simulink model "sm_pump_triplex"  (R2025a)
settings: Solver=VariableStepAuto  StartTime=0.0  StopTime=1.5  RelTol=1e-3  EnableMultiTasking=on
undefined symbols (not defined in the file): pOut_Init_WKSP, smiData, TRP_Par, X, Y, Z
libraries: sm_lib x43, fl_lib x30, nesl_utility x11, simulink x10, SimscapeFluids_lib x3, sm_pump_triplex_lib x3, ee_lib x2, Multibody_Multiphysics_Lib x1
(part 1 of 3)
CloseFcn:
  | try,close(h1_sm_pump_triplex),end
  | clear h1_sm_pump_triplex
  | try,close(h2_sm_pump_triplex),end
  | clear h2_sm_pump_triplex
  | try,close(h3_sm_pump_triplex),end
  | clear h3_sm_pump_triplex
  | try,close(h4_sm_pump_triplex),end
  | clear h4_sm_pump_triplex
  | try,close(h5_sm_pump_triplex),end
  | clear h5_sm_pump_triplex
  | try,close(h6_sm_pump_triplex),end
  | clear h6_sm_pump_triplex
  | try,close(h7_sm_pump_triplex),end
  | clear h7_sm_pump_triplex
  | 
  | clear simlog_sm_pump_triplex
  | clear logsout_sm_pump_triplex
Description:
  | Triplex Pump with Faults
  | 
  | Copyright 2017-2025 The MathWorks, Inc.
settings Model: Creator=smiller  LastModifiedBy=smiller
settings SolverCC: AlgebraicLoopSolver=TrustRegion
settings DataIOCC: InitialState=sm_pump_triplex_xFinal_steady_no_fault  LimitDataPoints=on  MaxDataPoints=20000  ReturnWorkspaceOutputs=off  SignalLoggingName=logsout_sm_pump_triplex
settings OptimizationCC: ReuseModelBlockBuffer=off  LifeSpan=inf
settings DebuggingCC: AlgebraicLoopMsg=error  UnconnectedInputMsg=warning  UnconnectedOutputMsg=warning  UnconnectedLineMsg=warning  AllowSymbolicDim=off  PregeneratedLibrarySubsystemCodeDiagnostic=none  SFUnexpectedBacktrackingDiag=warning  SFNoUnconditionalDefaultTransitionDiag=warning  SFExecutionAtInitializationDiag=none  ArithmeticOperatorsInVariantConditions=warning
settings ModelReferenceCC: EnableRefExpFcnMdlSchedulingChecks=on
settings SFSimCC: SimUseLocalCustomCode=off  CustomCodeUndefinedFunction=UseInterfaceOnly
settings RTWCC: RTWUseLocalCustomCode=off  GPUComputeCapability=3.5  DLArmComputeVersion=19.05
settings CodeAppCC: StateflowObjectComments=on
settings GRTTargetCC: TargetLangStandard=C89/C90 (ANSI)
settings ConfigComp: CovMetricSettings=dw  CovSaveCumulativeToWorkspaceVar=on  CovSaveSingleToWorkspaceVar=on  CovExternalEMLEnable=off  CovSFcnEnable=off
settings SimscapeCC: SimscapeNominalValues="[{\"value\":\"10\",\"unit\":\"V\"},{\"value\":\"1\",\"unit\":\"A\"},{\"value\":\"10\",\"unit\":\"N*m\"},{\"value\":\"10\",\"unit\":\"bar\"},{\"value\":\"100\",\"unit\":\"kJ/kg\"},{\"value\":\"1\",\"unit\":\"kW\"},{\"value\":\"300\",\"unit\":\"K\"},{\"value\":\"100\",\"unit\":\"cm^3/s\"},{\"value\":\"1\",\"unit\":\"kN\"},{\"value\":\"1\",\"unit\":\"g/cm^3\"},{\"value\":\"1\",\"unit\":\"l\"},{\"value\":\"1\",\"unit\":\"cm^2\"},{\"value\":\"60\",\"unit\":\"Hz\"}]"  SimscapeLogType=all  SimscapeLogSimulationStatistics=on  SimscapeLogName=simlog_sm_pump_triplex  SimscapeLogDataHistory=20000.0  SimscapeOperatingPoint=sm_pump_triplex_op_steady_no_fault
settings ConfigurationSet: Description=SimMechanics 2G
settings DiagnosticsConfigSet: SimMechanicsUnsatisfiedHighPriorityTargets=none
settings ExplorerConfigSet: InternalSimMechanicsExplorerSettings="<ExplorerConfiguration><canonicalview>default</canonicalview><AnimationSetting><BasePlaybackSpeed>1.0</BasePlaybackSpeed><PlaybackSpeedFactor>0.03125</PlaybackSpeedFactor></AnimationSetting><TilePanel><TileInfo><Tiles Columns=\"1\" Count=\"1\" Rows=\"1\"><Column Weight=\"1\"/><Row Weight=\"1\"/><Tile Height=\"1\" Width=\"1\" X=\"0\" Y=\"0\"/></Tiles></TileInfo><SceneInfo><SceneViewer><BGColor><R>1</R><G>1</G><B>1</B></BGColor><Camera><DoPerspective>off</DoPerspective><Position><X>0.719109619911456499</X><Y>0.503364840615347697</Y><Z>-0.352088882323819741</Z></Position><Center><X>-0.0103509884654956197</X><Y>-0.00162371159480578786</Y><Z>0.109293586960634348</Z></Center><Up><X>-0.420672049294932404</X><Y>0.863070110116374023</Y><Z>0.279544293387851028</Z></Up><ViewLimDist>1</ViewLimDist><YLim>0.144361463636159898</YLim><XLim>0.224724626591512072</XLim></Camera></SceneViewer></SceneInfo></TilePanel><MechEditorPanel><Cameras/><GfxPanelCameraMap/><VideoCreator><PlaybackSpeedRatio>1.0</PlaybackSpeedRatio><FrameRate>30</FrameRate><VideoFormat>Motion JPEG AVI</VideoFormat><FrameSize>auto</FrameSize></VideoCreator></MechEditorPanel></ExplorerConfiguration>"

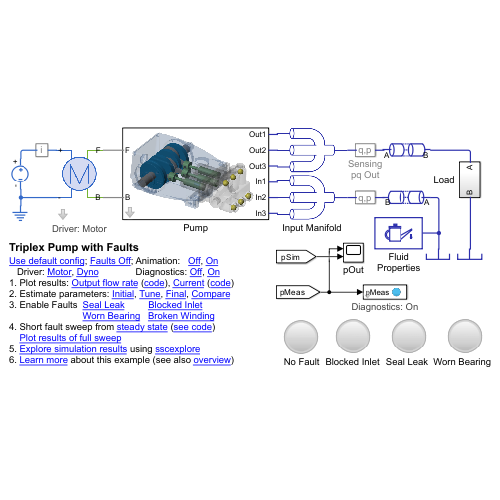
[thumbnail: Simulink's stored preview of the top-level diagram]
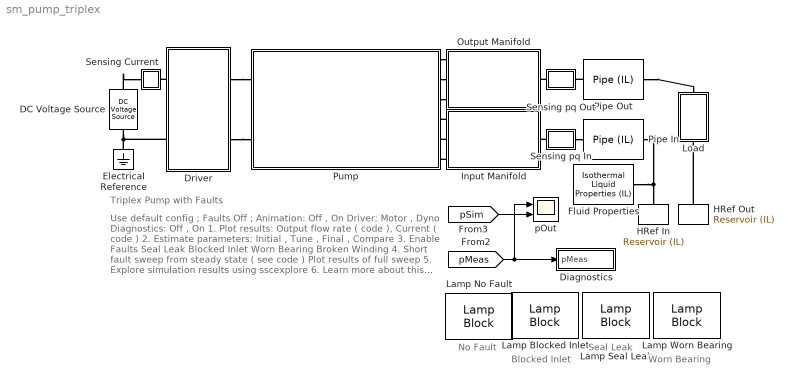
== system sm_pump_triplex ==
  note: No Fault
  note: Triplex Pump with Faults
  note: Use default config ; Faults Off ; Animation: Off , On
      | Driver: Motor , Dyno Diagnostics: Off , On
      | 1. Plot results: Output flow rate ( code ), Current ( code )
      | 2. Estimate parameters: Initial , Tune , Final , Compare
      | 3. Enable Faults Seal Leak Blocked Inlet
      | Worn Bearing Broken Winding
      | 4. Short fault sweep from steady state ( see code )
      | Plot results of full sweep
      | 5. Explore simulation results using sscexplore
      | 6. Learn more about this example (see also overview )
  note: Blocked Inlet
  note: Seal Leak
  note: Worn Bearing
  DC Voltage Source : ee_lib/Additional Components/SPICE Sources/DC Voltage Source  DC=24 V
  Diagnostics : Subsystem  mask{popup_fault_diagnostics=On, time_steady_state=1.4}
      mask prompts: popup_fault_diagnostics "Fault Diagnostics"; time_steady_state "Time to Steady State (s)"
      mask init:
      | set_param([gcb '/Diagnostics'],'OverrideUsingVariant',...
      |     get_param(gcb,'popup_fault_diagnostics'));
      settings: AttributesFormatString=Diagnostics: %<popup_fault_diagnostics>
      mask TypeOptions popup_fault_diagnostics: Off | On
      mask Callback popup_fault_diagnostics:
      | maskObj = Simulink.Mask.get(gcb);
      | timss_h = maskObj.getParameter('time_steady_state');
      | if (strcmp(get_param(gcb,'popup_fault_diagnostics'),'Off'))
      |     timss_h.Visible = 'off';
      | elseif (strcmp(get_param(gcb,'popup_fault_diagnostics'),'On'))
      |     timss_h.Visible = 'on';
      | end
      | clear maskObj timss_h
      mask Display:
      | if(strcmp(get_param(gcb,'popup_fault_diagnostics'),'On'))
      |     image('sm_pump_triplex_diagnostic_On_IMAGE.png');
      | else
      |     image('sm_pump_triplex_diagnostic_Off_IMAGE.png');
      | end
  Driver : Subsystem  Tag=PublishSubsystem  VariantControl=Electric  mask(Motor and Motor Driver){popup_driver_type=Motor, winding_fault_enable_P=Off, winding_fault_enable=On}
      mask prompts: popup_driver_type "Driver"; winding_fault_enable_P "Winding Fault"
      mask help: Model abstracts the torque-speed behavior of the combined motor and motor driver. Electric and control parameters are specified on blocks within the subsystem. The winding fault models a broken winding. When enabled, motor torque is set to 0 when the shaft angle is between 240 and 360 degrees (one-third of a shaft rotation).
      mask init:
      | curblk = gcb;
      | if(popup_driver_type==1)
      |     set_param([curblk '/Driver'],'OverrideUsingVariant','Motor');
      |     if(winding_fault_enable_P==1)
      |         set_param([curblk '/Driver/Motor'],'winding_fault_enable','Off');
      |     elseif(winding_fault_enable_P==2)
      |         set_param([curblk '/Driver/Motor'],'winding_fault_enable','On');
      |     end
      | elseif(popup_driver_type==2)
      |     set_param([curblk '/Driver'],'OverrideUsingVariant','Dyno');
      | end
      settings: AttributesFormatString=Driver: %<popup_driver_type>
      mask TypeOptions popup_driver_type: Motor | Dyno
      mask Callback popup_driver_type:
      | maskObj = Simulink.Mask.get(gcb);
      | windfault_h = maskObj.getParameter('winding_fault_enable_P');
      | if (strcmp(get_param(gcb,'popup_driver_type'),'Dyno'))
      |     windfault_h.Visible = 'off';
      | elseif (strcmp(get_param(gcb,'popup_driver_type'),'Motor'))
      |     windfault_h.Visible = 'on';
      | end
      | clear maskObj windfault_h
      mask TypeOptions winding_fault_enable_P: Off | On
      mask Display:
      | curblk = gcb;
      | if(strcmp(get_param(curblk,'popup_driver_type'),'Motor'))
      |     image('sm_pump_triplex_driverMotor_IMAGE.png');
      |     if(strcmp(get_param(curblk,'winding_fault_enable_P'),'On'))
      |         color('red');
      |         plot([0.85 0.6],[1.1 0.9])
      |         plot([0.6 0.85],[1.1 0.9])
      |         % Plot points to set plot range
      |         color('white');plot(1.2,2.4);plot(-1.2,-2.4)
      |         color('black');
      |     end
      | else
      |     image('sm_pump_triplex_driverDyno_IMAGE.png');
      | end
  Electrical Reference : fl_lib/Electrical/Electrical Elements/Electrical Reference
  Fluid Properties : fl_lib/Isothermal Liquid/Utilities/Isothermal Liquid Properties (IL)  rho_L_atm=851.6 kg/m^3  bulk_modulus_model=foundation.enum.bulk_modulus_model.const  beta_gain=6  beta_L_atm=1.46696e+09 Pa  nu_atm=(97.6333)*(1) cSt  p_atm=0.101325 MPa  p_min=1 Pa  properties_range_check=simscape.enum.assert.action.error  air_fraction=0.005  polytropic_index=1.0  rho_g_atm=1.225 kg/m^3  air_dissolution_model=simscape.enum.onoff.off  p_crit=3 MPa
      settings: LibrarySourceBlock=sh_lib/Hydraulic Utilities/Hydraulic Fluid
  HRef In : fl_lib/Isothermal Liquid/Elements/Reservoir (IL)  reservoir_type=foundation.enum.constant_controlled.constant  pressure_spec=foundation.enum.pressure_spec.atmospheric  reservoir_pressure=0.101325 MPa
      settings: LibrarySourceBlock=fl_lib/Hydraulic/Hydraulic Elements/Hydraulic Reference
  HRef Out : fl_lib/Isothermal Liquid/Elements/Reservoir (IL)  reservoir_type=foundation.enum.constant_controlled.constant  pressure_spec=foundation.enum.pressure_spec.atmospheric  reservoir_pressure=0.101325 MPa
      settings: LibrarySourceBlock=fl_lib/Hydraulic/Hydraulic Elements/Hydraulic Reference
  Input Manifold : Subsystem
      mask Display: image('sm_pump_triplex_Manifold_IMAGE.png');
  Lamp Blocked Inlet : LampBlock  LabelPosition=Hide  DefaultColor=[200.0, 200.0, 200.0]
  Lamp No Fault : LampBlock  LabelPosition=Hide  DefaultColor=[200.0, 200.0, 200.0]
  Lamp Seal Leak : LampBlock  LabelPosition=Hide  DefaultColor=[200.0, 200.0, 200.0]
  Lamp Worn Bearing : LampBlock  LabelPosition=Hide  DefaultColor=[200.0, 200.0, 200.0]
  Load : Subsystem
  Output Manifold : Subsystem
      mask Display: image('sm_pump_triplex_Manifold_IMAGE.png');
  Pipe In : SimscapeFluids_lib/Isothermal Liquid/Pipes & Fittings/Pipe (IL)  dynamic_compressibility=true  inertia=false  num_segments=1  pipe_length=5 m  cross_section_geometry=fluids.isothermal_liquid.pipes_fittings.enum.cross_section_geometry.circular  pipe_diameter=0.03 m  pipe_inner_diameter=0.05 m  pipe_outer_diameter=0.1 m  pipe_width=0.1 m  pipe_height=0.1 m  pipe_major_axis=0.1 m  pipe_minor_axis=0.05 m  pipe_side=0.1 m  pipe_angle=30 deg  pipe_area=1e-4 m^2  Dh=1.12e-2 m  elevation_spec=foundation.enum.constant_variable.constant  elevation_gain=0 m  gravity_spec=foundation.enum.constant_variable.constant  g=9.81 m/s^2  pressure_loss_spec=fluids.isothermal_liquid.pipes_fittings.enum.pressure_loss_spec.haaland  mdot_nominal=[.1, 1] kg/s  p_diff_nominal=[.001, .01] MPa  mdot_threshold=1e-6 kg/s  local_pressure_loss_spec=fluids.isothermal_liquid.pipes_fittings.enum.local_loss_spec.aggregate_length  length_add=1 m  loss_coefficient=0.1  roughness_spec=fluids.isothermal_liquid.pipes_fittings.enum.roughness_spec.custom  roughness=15e-6 m  Re_friction_TLU=[400, 1000, 1500, 3000, 4000, 6000, 10000, 20000, 40000, 60000, 100000, 100000000]  friction_factor_TLU=[.264, .112, .071, .0417, .0387, .0268, .025, .0232, .0226, .022, .0214, .0214]  Re_lam=2000  Re_tur=4000  shape_factor=64  pipe_wall_spec=fluids.isothermal_liquid.pipes_fittings.enum.wall_spec.rigid  vol_expansion_spec=fluids.isothermal_liquid.pipes_fittings.enum.vol_expansion_spec.area  area_pressure_gain=1e-6 m^2/MPa  static_pressure_TLU=[.1, 1] MPa  area_pressure_gain_TLU=[1e-05, 1.1e-05] m^2  material_behavior_spec=fluids.isothermal_liquid.pipes_fittings.enum.PipeMaterialBehavior.Linear  diameter_pressure_gain=2e-12 m/Pa  wall_thickness=0.05 m  elastic_modulus=69 GPa  stress_TLU=[276, 310] MPa  strain_TLU=[.004, .02]  stress_assert_action=simscape.enum.assert.action.none  stress_max=400 MPa  poisson_ratio=0.33  wall_time_constant=0.01 s  p0=0 + 101325 Pa  mdot0=0 kg/s
      settings: LibrarySourceBlock=sh_lib/Pipelines/Hydraulic Pipeline  InternalSimscapePortConfiguration="{\"Bottom\":[],\"Left\":[{\"id\":\"A\",\"label\":\"A\",\"type\":\"foundation.isothermal_liquid.isothermal_liquid\"}],\"Right\":[{\"id\":\"B\",\"label\":\"B\",\"type\":\"foundation.isothermal_liquid.isothermal_liquid\"}],\"Top\":[]}"
  Pipe Out : SimscapeFluids_lib/Isothermal Liquid/Pipes & Fittings/Pipe (IL)  dynamic_compressibility=true  inertia=false  num_segments=1  pipe_length=5 m  cross_section_geometry=fluids.isothermal_liquid.pipes_fittings.enum.cross_section_geometry.circular  pipe_diameter=0.03 m  pipe_inner_diameter=0.05 m  pipe_outer_diameter=0.1 m  pipe_width=0.1 m  pipe_height=0.1 m  pipe_major_axis=0.1 m  pipe_minor_axis=0.05 m  pipe_side=0.1 m  pipe_angle=30 deg  pipe_area=1e-4 m^2  Dh=1.12e-2 m  elevation_spec=foundation.enum.constant_variable.constant  elevation_gain=0 m  gravity_spec=foundation.enum.constant_variable.constant  g=9.81 m/s^2  pressure_loss_spec=fluids.isothermal_liquid.pipes_fittings.enum.pressure_loss_spec.haaland  mdot_nominal=[.1, 1] kg/s  p_diff_nominal=[.001, .01] MPa  mdot_threshold=1e-6 kg/s  local_pressure_loss_spec=fluids.isothermal_liquid.pipes_fittings.enum.local_loss_spec.aggregate_length  length_add=1 m  loss_coefficient=0.1  roughness_spec=fluids.isothermal_liquid.pipes_fittings.enum.roughness_spec.custom  roughness=15e-6 m  Re_friction_TLU=[400, 1000, 1500, 3000, 4000, 6000, 10000, 20000, 40000, 60000, 100000, 100000000]  friction_factor_TLU=[.264, .112, .071, .0417, .0387, .0268, .025, .0232, .0226, .022, .0214, .0214]  Re_lam=2000  Re_tur=4000  shape_factor=64  pipe_wall_spec=fluids.isothermal_liquid.pipes_fittings.enum.wall_spec.rigid  vol_expansion_spec=fluids.isothermal_liquid.pipes_fittings.enum.vol_expansion_spec.area  area_pressure_gain=1e-6 m^2/MPa  static_pressure_TLU=[.1, 1] MPa  area_pressure_gain_TLU=[1e-05, 1.1e-05] m^2  material_behavior_spec=fluids.isothermal_liquid.pipes_fittings.enum.PipeMaterialBehavior.Linear  diameter_pressure_gain=2e-12 m/Pa  wall_thickness=0.05 m  elastic_modulus=69 GPa  stress_TLU=[276, 310] MPa  strain_TLU=[.004, .02]  stress_assert_action=simscape.enum.assert.action.none  stress_max=400 MPa  poisson_ratio=0.33  wall_time_constant=0.01 s  p0=pOut_Init_WKSP + 1.01325 bar  mdot0=0 kg/s
      settings: LibrarySourceBlock=sh_lib/Pipelines/Hydraulic Pipeline  InternalSimscapePortConfiguration="{\"Bottom\":[],\"Left\":[{\"id\":\"A\",\"label\":\"A\",\"type\":\"foundation.isothermal_liquid.isothermal_liquid\"}],\"Right\":[{\"id\":\"B\",\"label\":\"B\",\"type\":\"foundation.isothermal_liquid.isothermal_liquid\"}],\"Top\":[]}"
  Pump : Subsystem  Tag=PublishSubsystem  mask(Triplex Pump with Faults){cyl_gap_P=TRP_Par.Cylinder.gap, cyl_rad_out_P=TRP_Par.Cylinder.rad_outer, cyl_len_P=TRP_Par.Cylinder.len, cyl_stroke_P=TRP_Par.Cylinder.stroke, cyl_frict_brkway_frc_P=TRP_Par.Cylinder.Friction.BrkFrc, cyl_frict_brkway_vel_P=TRP_Par.Cylinder.Friction.BrkVel, cyl_frict_col_frc_P=TRP_Par.Cylinder.Friction.ColFrc, cyl_frict_visc_coef_P=TRP_Par.Cylinder.Friction.ViscCo, cyl_rho_P=TRP_Par.Cylinder.rho, cyl_clr_P=TRP_Par.Cylinder.clr, cyl_opc_P=TRP_Par.Cylinder.opc, plgB_len_P=TRP_Par.Plunger.len, plgB_rad_P=TRP_Par.Plunger.rad, stem_len_P=TRP_Par.Stem.len, stem_rad_P=TRP_Par.Stem.rad, pin_len_P=TRP_Par.Pin.len, pin_rad_P=TRP_Par.Pin.rad, cup_rad_out_P=TRP_Par.StemCup.rad, cup_thk_P=TRP_Par.StemCup.wall, cup_len_P=TRP_Par.StemCup.len, cup_pinOffset_P=TRP_Par.StemCup.pinOffset, plg_rho_P=TRP_Par.Plunger.rho, plg_clr_P=TRP_Par.Plunger.clr, plg_opc_P=TRP_Par.Plunger.opc, conrod_len_P=TRP_Par.ConRod.len, conrod_web_widP_P=TRP_Par.ConRod.W1, conrod_web_widC_P=TRP_Par.ConRod.W2, conrod_ringC_wid_P=TRP_Par.ConRod.R2.width, conrod_ringP_wid_P=TRP_Par.ConRod.R1.width, crank_shaft_rad_P=TRP_Par.Crank.Shaft.rad, conrod_thk_P=TRP_Par.ConRod.hei, conrod_rho_P=TRP_Par.ConRod.rho, conrod_clr_P=TRP_Par.ConRod.clr, conrod_opc_P=TRP_Par.ConRod.opc, chkv_in_maxA_P=TRP_Par.Check_Valve.In.Max_Area, chkv_out_maxA_P=TRP_Par.Check_Valve.Out.Max_Area, chkv_press_set_popup_P=Set in Mask, chkv_in_crkP_P=TRP_Par.Check_Valve.In.Crack_Pr, chkv_out_crkP_P=TRP_Par.Check_Valve.Out.Crack_Pr, chkv_in_maxOpenP_P=TRP_Par.Check_Valve.In.Max_Open_Pr, chkv_out_maxOpenP_P=TRP_Par.Check_Valve.Out.Max_Open_Pr, chkv_vis_popup_P=On, chkv_vis_rad_in_P=TRP_Par.Check_Valve.In.Vis.rad, chkv_vis_rad_out_P=TRP_Par.Check_Valve.Out.Vis.rad, chkv_vis_clr_in_P=TRP_Par.Check_Valve.In.Vis.clr, chkv_vis_clr_out_P=TRP_Par.Check_Valve.Out.Vis.clr, shaft_rad_P=TRP_Par.Crank.Shaft.rad, shaft_len_P=TRP_Par.Crank.Shaft.len, web_rad_P=TRP_Par.Crank.Cam.rad, web_len_P=TRP_Par.Crank.Cam.wid, motor_shaft_rad_P=TRP_Par.Motor.Shaft.rad, motor_shaft_len_P=TRP_Par.Motor.Shaft.len, shaft_pos_P=TRP_Par.Crank.Shaft.pos, crank_rho_P=TRP_Par.Crank.rho, bearing_visc_frict=TRP_Par.Crank.Bearing.b, crank_clr_P=TRP_Par.Crank.Cam.clr, motor_shaft_clr_P=TRP_Par.Motor.Shaft.clr, crank_opc_P=TRP_Par.Crank.Cam.opc, crank_ax_offset=TRP_Par.Crank.axoffset, bearing_sep=TRP_Par.Crank.Bearing_sep, housing_clr=TRP_Par.Housing.clr, housing_opc=TRP_Par.Housing.opc, manifold_clr=TRP_Par.Manifold.clr, manifold_opc=TRP_Par.Manifold.opc, leak_cyl1_popup=Off, leak_cyl2_popup=Off, leak_cyl3_popup=Off, leak_cyl1_area=TRP_Par.Check_Valve.In.Max_Area*0.03, leak_cyl2_area=TRP_Par.Check_Valve.In.Max_Area*0.03, leak_cyl3_area=TRP_Par.Check_Valve.In.Max_Area*0.03, block_in_cyl1_popup=Off, block_in_cyl2_popup=Off, block_in_cyl3_popup=Off, block_in_cyl1_factor=0.5, block_in_cyl2_factor=0.5, block_in_cyl3_factor=0.5, bearing_fault_popup=Off, bearing_fault_frict=3e-4, seal_leak_vis_len_P=TRP_Par.Seal_Leak.len, seal_leak_vis_rad_P=TRP_Par.Seal_Leak.rad, seal_leak_vis_clr_P=TRP_Par.Seal_Leak.clr, inlet_obstr_len_P=TRP_Par.Manifold.Inlet.obstr.len, inlet_obstr_rad_P=TRP_Par.Manifold.Inlet.rad, inlet_obstr_clr_P=TRP_Par.Manifold.Inlet.obstr.clr, bearing_fault_vis_len=TRP_Par.Crank.Bearing_Fault.len, bearing_fault_vis_rad=TRP_Par.Crank.Bearing_Fault.rad, bearing_fault_vis_clr=TRP_Par.Crank.Bearing_Fault.clr, bearing_fault_vis_opc=0}
      mask prompts: cyl_gap_P "Gap (m)"; cyl_rad_out_P "Outer Radius (m)"; cyl_len_P "Length (m)"; cyl_stroke_P "Stroke (m)"; cyl_frict_brkway_frc_P "Breakaway Friction Force (N)"; cyl_frict_brkway_vel_P "Breakaway Friction Velocity (m/s)"; cyl_frict_col_frc_P "Coulomb Friction Force (N)"; cyl_frict_visc_coef_P "Viscous Friction Coeff (N/(m/s))"; cyl_rho_P "Density (kg/m^3)"; cyl_clr_P "Color [RGB]"; cyl_opc_P "Opacity (0-1)"; cup_rad_out_P "Outer Radius (m)"; cup_thk_P "Wall Thickness (m)"; cup_len_P "Length(m)"; cup_pinOffset_P "Pin Offset (m)"; plg_rho_P "Density (kg/m^3)"; plg_clr_P "Color [RGB]"; plg_opc_P "Opacity (0-1)"; conrod_len_P "Length, center-center (m)"; conrod_web_widP_P "Width, pin end (m)"; conrod_web_widC_P "Width, crank end (m)"; conrod_ringC_wid_P "Crank Ring Width (m)"; conrod_ringP_wid_P "Pin Ring Width (m)"; crank_shaft_rad_P "Crank Shaft Radius (m)"; conrod_thk_P "Thickness (m)"; conrod_rho_P "Density (kg/m^3)"; conrod_clr_P "Color [RGB]"; conrod_opc_P "Opacity (0-1)"; chkv_press_set_popup_P "Pressure Settings"; chkv_vis_popup_P "Valve Visualization"; shaft_pos_P "Crankpin Axis Offset (m)"; crank_rho_P "Density (kg/m^3)"; bearing_visc_frict "Bearing Viscous Friction (N*m/(deg/s))"; crank_clr_P "Crank Color [RGB]"; motor_shaft_clr_P "Motor Shaft Color [RGB]"; crank_opc_P "Opacity (0-1)"; crank_ax_offset "Crankshaft Axis Offset [XYZ] (m)"; bearing_sep "Bearing Separation (m)"; housing_clr "Housing Color [RGB]"; housing_opc "Housing Opacity (0-1)"; manifold_clr "Manifold Color [RGB]"; manifold_opc "Manifold Opacity (0-1)"; leak_cyl1_area "Plunger 1 Leak Area (m^2)"; leak_cyl2_area "Plunger 2 Leak Area (m^2)"; leak_cyl3_area "Plunger 3 Leak Area (m^2)"; block_in_cyl1_factor "Blocked Inlet 1: Area Factor (0-1)"; block_in_cyl2_factor "Blocked Inlet 2: Area Factor (0-1)"; block_in_cyl3_factor "Blocked Inlet 3: Area Factor (0-1)"; bearing_fault_popup "Bearing Wear"; bearing_fault_frict "Additional Friction (N*m/(deg/s))"; seal_leak_vis_len_P "Length (m)"; seal_leak_vis_rad_P "Radius (m)"; seal_leak_vis_clr_P "Color [RGB]"; inlet_obstr_len_P "Length (m)"; inlet_obstr_rad_P "Radius (m)"; inlet_obstr_clr_P "Color [RGB]"; bearing_fault_vis_len "Length (m)"; bearing_fault_vis_rad "Radius (m)"; bearing_fault_vis_clr "Color [RGB]"; bearing_fault_vis_opc "Opacity (0-1)"
      mask help: Models a triplex pump. Three hydraulic plungers are connected to a crankshaft. Hydraulic and mechanical faults can be enabled on the Faults tab.
      mask init:
      | % -- Configure Plunger Faults
      | set_param([gcb '/Plunger 1'],'leak_cyl_popup',...
      |     get_param(gcb,'leak_cyl1_popup'));
      | set_param([gcb '/Plunger 2'],'leak_cyl_popup',...
      |     get_param(gcb,'leak_cyl2_popup'));
      | set_param([gcb '/Plunger 3'],'leak_cyl_popup',...
      |     get_param(gcb,'leak_cyl3_popup'));
      | 
      | set_param([gcb '/Plunger 1'],'block_in_popup',...
      |     get_param(gcb,'block_in_cyl1_popup'));
      | set_param([gcb '/Plunger 2'],'block_in_popup',...
      |     get_param(gcb,'block_in_cyl2_popup'));
      | set_param([gcb '/Plunger 3'],'block_in_popup',...
      |     get_param(gcb,'block_in_cyl3_popup'));
      | 
      | % -- Set valve visualization
      | set_param([gcb '/Plunger 1'],'chkv_vis_popup',...
      |     get_param(gcb,'chkv_vis_popup_P'));
      | set_param([gcb '/Plunger 2'],'chkv_vis_popup',...
      |     get_param(gcb,'chkv_vis_popup_P'));
      | set_param([gcb '/Plunger 3'],'chkv_vis_popup',...
      |     get_param(gcb,'chkv_vis_popup_P'));
      | 
      | % -- Configure bearing fault
      | if(bearing_fault_popup==1)
      |     set_param([gcb '/Crank Bearing'],...
      |         'DampingCoefficient','bearing_visc_frict',...
      |         'DampingCoefficient_conf','compiletime');
      |     bearing_fault_vis_opc = 0;
      | elseif(bearing_fault_popup==2)
      |     set_param([gcb '/Crank Bearing'],...
      |         'DampingCoefficient','bearing_visc_frict+bearing_fault_frict',...
      |         'DampingCoefficient_conf','compiletime');
      |     bearing_fault_vis_opc = 1;
      | elseif(bearing_fault_popup==3)
      |     set_param([gcb '/Crank Bearing'],...
      |         'DampingCoefficient','bearing_visc_frict_WKSP+bearing_fault_frict_WKSP',...
      |         'DampingCoefficient_conf','runtime');
      |     bearing_fault_vis_opc = 1;
      | end
      | 
      | % -- Configure tuning option for pressure settings
      | set_param([gcb '/Plunger 1'],'chkv_press_set_popup',...
      |     get_param(gcb,'chkv_press_set_popup_P'));
      | set_param([gcb '/Plunger 2'],'chkv_press_set_popup',...
      |     get_param(gcb,'chkv_press_set_popup_P'));
      | set_param([gcb '/Plunger 3'],'chkv_press_set_popup',...
      |     get_param(gcb,'chkv_press_set_popup_P'));
      mask TypeOptions chkv_press_set_popup_P: Set in Mask | Tune at Run Time
      mask Callback chkv_press_set_popup_P:
      | maskObj = Simulink.Mask.get(gcb);
      | 
      | crPrP_h = maskObj.getDialogControl('text_open_crkP');
      | crMxP_h = maskObj.getDialogControl('text_open_maxOpenP');
      | crPIn_h = maskObj.getParameter('chkv_in_crkP_P');
      | crPOu_h = maskObj.getParameter('chkv_out_crkP_P');
      | mxPIn_h = maskObj.getParameter('chkv_in_maxOpenP_P');
      | mxPOu_h = maskObj.getParameter('chkv_out_maxOpenP_P');
      | 
      | allTxt_h = maskObj.getDialogControl('chkv_pres_set_all_tune_text');
      | 
      | temp_PressSetTune = get_param(gcb,'chkv_press_set_popup_P');
      | 
      | if (strcmp(temp_PressSetTune,'Set in Mask'))
      |     crPrP_h.Visible = 'on';
      |     crMxP_h.Visible = 'on';
      |     crPIn_h.Visible = 'on';
      |     crPOu_h.Visible = 'on';
      |     mxPIn_h.Visible = 'on';
      |     mxPOu_h.Visible = 'on';
      |     allTxt_h.Visible = 'off';
      |     outTxt_h.Visible = 'off';
      | else
      |     crPrP_h.Visible = 'off';
      |     crMxP_h.Visible = 'off';
      |     crPIn_h.Visible = 'off';
      |     crPOu_h.Visible = 'off';
      |     mxPIn_h.Visible = 'off';
      |     mxPOu_h.Visible = 'off';
      |     allTxt_h.Visible = 'on';
      |     outTxt_h.Visible = 'on';
      | end
      | clear maskObj temp_PressSetTune
      | clear crPrP_h crMxP_h crPIn_h crPOu_h mxPIn_h mxPOu_h
      | clear allTxt_h
      mask TypeOptions chkv_vis_popup_P: Off | On
      mask TypeOptions leak_cyl1_popup: Off | On | On, Run Time
      mask Callback leak_cyl1_popup:
      | maskObj = Simulink.Mask.get(gcb);
      | leak_cyl1_area_h = maskObj.getParameter('leak_cyl1_area');
      | leak_cyl1_text_h = maskObj.getDialogControl('leak_cyl1_tune_text');
      | if (strcmp(get_param(gcb,'leak_cyl1_popup'),'Off'))
      |     leak_cyl1_area_h.Visible = 'off';
      |     leak_cyl1_text_h.Visible = 'off';
      | elseif (strcmp(get_param(gcb,'leak_cyl1_popup'),'On'))
      |     leak_cyl1_area_h.Visible = 'on';
      |     leak_cyl1_text_h.Visible = 'off';
      | elseif (strcmp(get_param(gcb,'leak_cyl1_popup'),'On, Run Time'))
      |     leak_cyl1_area_h.Visible = 'off';
      |     leak_cyl1_text_h.Visible = 'on';
      | end
      | clear maskObj leak_cyl1_area_h leak_cyl1_text_h
      mask TypeOptions leak_cyl2_popup: Off | On | On, Run Time
      mask Callback leak_cyl2_popup:
      | maskObj = Simulink.Mask.get(gcb);
      | leak_cyl2_area_h = maskObj.getParameter('leak_cyl2_area');
      | leak_cyl2_text_h = maskObj.getDialogControl('leak_cyl2_tune_text');
      | if (strcmp(get_param(gcb,'leak_cyl2_popup'),'Off'))
      |     leak_cyl2_area_h.Visible = 'off';
      |     leak_cyl2_text_h.Visible = 'off';
      | elseif (strcmp(get_param(gcb,'leak_cyl2_popup'),'On'))
      |     leak_cyl2_area_h.Visible = 'on';
      |     leak_cyl2_text_h.Visible = 'off';
      | elseif (strcmp(get_param(gcb,'leak_cyl2_popup'),'On, Run Time'))
      |     leak_cyl2_area_h.Visible = 'off';
      |     leak_cyl2_text_h.Visible = 'on';
      | end
      | clear maskObj leak_cyl2_area_h leak_cyl2_text_h
      mask TypeOptions leak_cyl3_popup: Off | On | On, Run Time
      mask Callback leak_cyl3_popup:
      | maskObj = Simulink.Mask.get(gcb);
      | leak_cyl3_area_h = maskObj.getParameter('leak_cyl3_area');
      | leak_cyl3_text_h = maskObj.getDialogControl('leak_cyl3_tune_text');
      | if (strcmp(get_param(gcb,'leak_cyl3_popup'),'Off'))
      |     leak_cyl3_area_h.Visible = 'off';
      |     leak_cyl3_text_h.Visible = 'off';
      | elseif (strcmp(get_param(gcb,'leak_cyl3_popup'),'On'))
      |     leak_cyl3_area_h.Visible = 'on';
      |     leak_cyl3_text_h.Visible = 'off';
      | elseif (strcmp(get_param(gcb,'leak_cyl3_popup'),'On, Run Time'))
      |     leak_cyl3_area_h.Visible = 'off';
      |     leak_cyl3_text_h.Visible = 'on';
      | end
      | clear maskObj leak_cyl3_area_h leak_cyl3_text_h
      mask TypeOptions block_in_cyl1_popup: Off | On | On, Run Time
      mask Callback block_in_cyl1_popup:
      | maskObj = Simulink.Mask.get(gcb);
      | cyl_factor_h = maskObj.getParameter('block_in_cyl1_factor');
      | cyl_text_h = maskObj.getDialogControl('block_in_cyl1_tune_text');
      | tmp_block_in_cyl = get_param(gcb,'block_in_cyl1_popup');
      | 
      | if (strcmp(tmp_block_in_cyl,'Off'))
      |     cyl_factor_h.Visible = 'off';
      |     cyl_text_h.Visible = 'off';
      | elseif (strcmp(tmp_block_in_cyl,'On'))
      |     cyl_factor_h.Visible = 'on';
      |     cyl_text_h.Visible = 'off';
      | elseif (strcmp(tmp_block_in_cyl,'On, Run Time'))
      |     cyl_factor_h.Visible = 'off';
      |     cyl_text_h.Visible = 'on';
      | end
      | clear maskObj tmp_block_in_cyl cyl_factor_h cyl_text_h
      mask TypeOptions block_in_cyl2_popup: Off | On | On, Run Time
      mask Callback block_in_cyl2_popup:
      | maskObj = Simulink.Mask.get(gcb);
      | cyl_factor_h = maskObj.getParameter('block_in_cyl2_factor');
      | cyl_text_h = maskObj.getDialogControl('block_in_cyl2_tune_text');
      | tmp_block_in_cyl = get_param(gcb,'block_in_cyl2_popup');
      | 
      | if (strcmp(tmp_block_in_cyl,'Off'))
      |     cyl_factor_h.Visible = 'off';
      |     cyl_text_h.Visible = 'off';
      | elseif (strcmp(tmp_block_in_cyl,'On'))
      |     cyl_factor_h.Visible = 'on';
      |     cyl_text_h.Visible = 'off';
      | elseif (strcmp(tmp_block_in_cyl,'On, Run Time'))
      |     cyl_factor_h.Visible = 'off';
      |     cyl_text_h.Visible = 'on';
      | end
      | clear maskObj tmp_block_in_cyl cyl_factor_h cyl_text_h
      mask TypeOptions block_in_cyl3_popup: Off | On | On, Run Time
      mask Callback block_in_cyl3_popup:
      | maskObj = Simulink.Mask.get(gcb);
      | cyl_factor_h = maskObj.getParameter('block_in_cyl3_factor');
      | cyl_text_h = maskObj.getDialogControl('block_in_cyl3_tune_text');
      | tmp_block_in_cyl = get_param(gcb,'block_in_cyl3_popup');
      | 
      | if (strcmp(tmp_block_in_cyl,'Off'))
      |     cyl_factor_h.Visible = 'off';
      |     cyl_text_h.Visible = 'off';
      | elseif (strcmp(tmp_block_in_cyl,'On'))
      |     cyl_factor_h.Visible = 'on';
      |     cyl_text_h.Visible = 'off';
      | elseif (strcmp(tmp_block_in_cyl,'On, Run Time'))
      |     cyl_factor_h.Visible = 'off';
      |     cyl_text_h.Visible = 'on';
      | end
      | clear maskObj tmp_block_in_cyl cyl_factor_h cyl_text_h
      mask TypeOptions bearing_fault_popup: Off | On | On, Run Time
      mask Callback bearing_fault_popup:
      | maskObj = Simulink.Mask.get(gcb);
      | bf_frict_h = maskObj.getParameter('bearing_fault_frict');
      | bf_text_h = maskObj.getDialogControl('bearing_fault_tune_text');
      | tmp_bearing_fault = get_param(gcb,'bearing_fault_popup');
      | 
      | if (strcmp(tmp_bearing_fault,'Off'))
      |     bf_frict_h.Visible = 'off';
      |     bf_text_h.Visible = 'off';
      | elseif (strcmp(tmp_bearing_fault,'On'))
      |     bf_frict_h.Visible = 'on';
      |     bf_text_h.Visible = 'off';
      | elseif (strcmp(tmp_bearing_fault,'On, Run Time'))
      |     bf_frict_h.Visible = 'off';
      |     bf_text_h.Visible = 'on';
      | end
      | clear maskObj tmp_bearing_fault bf_frict_h bf_text_h
      mask DialogControl tab_cylinder Prompt: Cyl.
      mask DialogControl cont_dims Prompt: Dimensions
      mask DialogControl cont_friction Prompt: Friction
      mask DialogControl cont_cyl_vis Prompt: Cylinder Visualization
      mask DialogControl tab_plunger Prompt: Plung.
      mask DialogControl text_length Prompt: Length (m)
      mask DialogControl text_radius Prompt: Radius (m)
      mask DialogControl text_base Prompt: Base
      mask DialogControl text_stem Prompt: Stem
      mask DialogControl text_pin Prompt: Pin
      mask DialogControl cont_cup Prompt: Cup
      mask DialogControl cont_plg_vis Prompt: Plunger Visualization
      mask DialogControl tab_conrod Prompt: Rod
      mask DialogControl cont_conrodWeb Prompt: Web
      mask DialogControl cont_conrodRings Prompt: Rings
      mask DialogControl cont_conrod_vis Prompt: Rod Visualization
      mask DialogControl tab_valves Prompt: Valve
      mask DialogControl text_open_inlet Prompt: Inlet
      mask DialogControl text_open_outlet Prompt: Outlet
      mask DialogControl text_open_maxA Prompt: Max Area (m)
      mask DialogControl text_open_crkP Prompt: Crack. Pr (Pa)
      mask DialogControl text_open_maxOpenP Prompt: Max Pr. (Pa)
      mask DialogControl chkv_pres_set_all_tune_text Prompt: Set >> chkv_all_crkP_WKSP, chkv_all_maxOpenP_WKSP
      mask DialogControl Container22 Prompt: Visualization Settings
      mask DialogControl text_valvis_inlet Prompt: Inlet
      mask DialogControl text_valvis_outlet Prompt: Outlet
      mask DialogControl text_valvis_rad Prompt: Radius (m)
      mask DialogControl text_valvis_clr Prompt: Color [RGB]
      mask DialogControl tab_crank Prompt: Crank
      mask DialogControl text_crank_rad Prompt: Radius (m)
      mask DialogControl text_crank_len Prompt: Length (m)
      mask DialogControl text_crankpin Prompt: Crankpin
      mask DialogControl text_web Prompt: Web
      mask DialogControl text_motor_shaft Prompt: Motor Shaft
      mask DialogControl cont_crank_vis Prompt: Crankshaft Visualization
      mask DialogControl tab_housing Prompt: Housing
      mask DialogControl cont_vis Prompt: Visualization
      mask DialogControl tab_faults Prompt: Fault
      mask DialogControl Control12 Prompt: Plunger 1
      mask DialogControl Control13 Prompt: Plunger 2
      mask DialogControl Control14 Prompt: Plunger 3
      mask DialogControl Control10 Prompt: Seal Leak
      mask DialogControl leak_cyl1_tune_text Prompt: Plunger 1:  Set >> leak_cyl_area_WKSP
      mask DialogControl leak_cyl2_tune_text Prompt: Plunger 2:  Set >> leak_cyl_area_WKSP
      mask DialogControl leak_cyl3_tune_text Prompt: Plunger 3:  Set >> leak_cyl_area_WKSP
      mask DialogControl Control19 Prompt: Blocked Inlet
      mask DialogControl block_in_cyl1_tune_text Prompt: Plunger 1: Set >> block_in_factor_WKSP, chkv_out_maxA_WKSP
      mask DialogControl block_in_cyl2_tune_text Prompt: Plunger 2: Set >> block_in_factor_WKSP, chkv_out_maxA_WKSP
      mask DialogControl block_in_cyl3_tune_text Prompt: Plunger 3: Set >> block_in_factor_WKSP, chkv_out_maxA_WKSP
      mask DialogControl bearing_fault_tune_text Prompt: Set >> bearing_visc_frict_WKSP, bearing_fault_frict_WKSP
      mask DialogControl cont_seal_leak_vis Prompt: Seal Leak Visualization
      mask DialogControl cont_blocked_line_vis Prompt: Blocked Line Visualization
      mask DialogControl cont_bearing_fault_vis Prompt: Bearing Fault Visualization
      mask Display:
      | if(strcmp(get_param(gcb,'chkv_vis_popup_P'),'On'))
      |     image('sm_pump_triplex_Pump_VisOn_IMAGE.png');
      | else
      |     image('sm_pump_triplex_Pump_VisOff_IMAGE.png');
      | end
      | color('white');
      | plot(0,0);
      | plot(659,412);
      | color('red');
      | if(~strcmp(get_param(gcb,'block_in_cyl3_popup'),'Off'))
      |     plot([510 530],[30 50]);
      |     plot([530 510],[30 50]);
      | end
      | if(~strcmp(get_param(gcb,'block_in_cyl2_popup'),'Off'))
      |     plot([540 560],[55 75]);
      |     plot([560 540],[55 75]);
      | end
      | if(~strcmp(get_param(gcb,'block_in_cyl1_popup'),'Off'))
      |     plot([575 595],[85 105]);
      |     plot([595 575],[85 105]);
      | end
      | if(~strcmp(get_param(gcb,'leak_cyl3_popup'),'Off'))
      |     plot([300 320],[155 175]);
      |     plot([320 300],[155 175]);
      | end
      | if(~strcmp(get_param(gcb,'leak_cyl2_popup'),'Off'))
      |     plot([335 355],[185 205]);
      |     plot([355 335],[185 205]);
      | end
      | if(~strcmp(get_param(gcb,'leak_cyl1_popup'),'Off'))
      |     plot([365 385],[215 235]);
      |     plot([385 365],[215 235]);
      | end
      | if(~strcmp(get_param(gcb,'bearing_fault_popup'),'Off'))
      |     plot([100 120],[185 205]);
      |     plot([120 100],[185 205]);
      | end
      | color('gray')
      | if(strcmp(get_param(gcb,'chkv_press_set_popup_P'),'Tune at Run Time'))
      |     plot([470 485 500 515]+60,[30 30 50 50]-10);
      | end
  Sensing Current : Subsystem
      mask Display: disp('i');
  Sensing pq In : Subsystem
      mask Display: disp('q,p');
  Sensing pq Out : Subsystem
      mask Display: disp('q,p');
  pOut : Scope  NumInputPorts=2
      settings: Title=Pump Output Pressure  ActiveDisplayYMinimum=6.95483  ActiveDisplayYMaximum=7.36166
  wires:
  [pMeas] -> pOut/1, Diagnostics/1(pMeas)
  [pSim] -> pOut/2
  connections:
  Input Manifold/LConn2 -- Pump/RConn5
  Input Manifold/LConn1 -- Pump/RConn4
  Input Manifold/LConn3 -- Pump/RConn6
  Pump/RConn1 -- Output Manifold/LConn1
  Pump/RConn2 -- Output Manifold/LConn2
  Pump/RConn3 -- Output Manifold/LConn3
  Sensing pq Out/LConn1 -- Output Manifold/RConn1
  DC Voltage Source/LConn1 -- Sensing Current/LConn1
  Driver/LConn2 -- Electrical Reference/LConn1 -- DC Voltage Source/RConn1
  Driver/LConn1 -- Sensing Current/RConn1
  Pipe Out/LConn1 -- Sensing pq Out/RConn1
  Pipe Out/RConn1 -- Load/LConn1
  HRef Out/LConn1 -- Load/RConn1
  Fluid Properties/RConn1 -- Pipe In/LConn1 -- HRef In/LConn1
  Sensing pq In/RConn1 -- Input Manifold/RConn1
  Sensing pq In/LConn1 -- Pipe In/RConn1
  Driver/RConn1 -- Pump/LConn1
  Driver/RConn2 -- Pump/LConn2

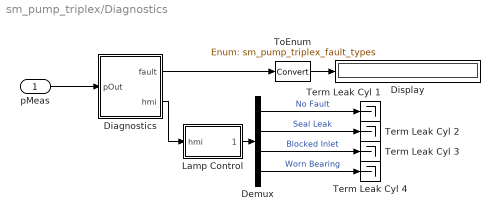
== system sm_pump_triplex/Diagnostics ==
  pMeas : Inport
  Demux : Demux
  Diagnostics : Subsystem  Variant=on  VariantControlMode=label  VariantControl=Variant1  LabelModeActiveChoice=On
  Display : Display
  Lamp Control : Subsystem
  Term Leak Cyl {1..4} (4 alike) : Terminator
  ToEnum : DataTypeConversion  OutDataTypeStr=Enum: sm_pump_triplex_fault_types  SaturateOnIntegerOverflow=off  RndMeth=Floor
  wires:
  Demux/1 -> Term Leak Cyl 1/1  "No Fault"
  Demux/3 -> Term Leak Cyl 3/1  "Blocked Inlet"
  Demux/2 -> Term Leak Cyl 2/1  "Seal Leak"
  Demux/4 -> Term Leak Cyl 4/1  "Worn Bearing"
  ToEnum/1 -> Display/1
  pMeas/1 -> Diagnostics/1("pOut ")
  Diagnostics/1(" fault") -> ToEnum/1
  Diagnostics/2(" hmi") -> Lamp Control/1(hmi)
  Lamp Control/1(lamps) -> Demux/1

== system sm_pump_triplex/Driver ==
  Driver : Subsystem  Variant=on  VariantControlMode=label  VariantControl=Variant1  LabelModeActiveChoice=Motor
      settings: AttributesFormatString=%<ActiveVariant>
  F : PMIOPort  Side=Right
  B : PMIOPort  Port=2  Side=Right
  + : PMIOPort  Port=3  Side=Left
  - : PMIOPort  Port=4  Side=Left
  connections:
  Driver/LConn1 -- +/RConn1
  Driver/LConn2 -- -/RConn1
  Driver/RConn1 -- F/RConn1
  Driver/RConn2 -- B/RConn1

== system sm_pump_triplex/Input Manifold ==
  Chamber : fl_lib/Isothermal Liquid/Elements/Constant Volume Chamber (IL)  volume=2e-4 m^3  p_I_specify=off  p_I_priority=High  p_I=0 + 101325 Pa  p_I_nominal_specify=off  p_I_nominal_value=1  p_I_nominal_unit=Pa
      settings: InternalSimscapePortConfiguration="{\"Bottom\":[],\"Left\":[{\"id\":\"A\",\"label\":\"A\",\"type\":\"foundation.isothermal_liquid.isothermal_liquid\"}],\"Right\":[],\"Top\":[]}"
      settings: LibrarySourceBlock=|
      | fl_lib/Hydraulic/Hydraulic Elements/Constant Volume
      | Hydraulic Chamber
  A : PMIOPort  Side=Right
  B1 : PMIOPort  Port=2  Side=Left
  B2 : PMIOPort  Port=3  Side=Left
  B3 : PMIOPort  Port=4  Side=Left
  connections:
  Chamber/LConn1 -- A/RConn1 -- B1/RConn1 -- B2/RConn1 -- B3/RConn1

== system sm_pump_triplex/Load ==
  Chamber : fl_lib/Isothermal Liquid/Elements/Constant Volume Chamber (IL)  volume=1e-4 m^3  p_I_specify=on  p_I_priority=High  p_I=pOut_Init_WKSP + 1.01325 bar  p_I_nominal_specify=off  p_I_nominal_value=1  p_I_nominal_unit=Pa
      settings: InternalSimscapePortConfiguration="{\"Bottom\":[],\"Left\":[{\"id\":\"A\",\"label\":\"A\",\"type\":\"foundation.isothermal_liquid.isothermal_liquid\"}],\"Right\":[],\"Top\":[]}"
      settings: LibrarySourceBlock=|
      | fl_lib/Hydraulic/Hydraulic Elements/Constant Volume
      | Hydraulic Chamber
  Orifice : SimscapeFluids_lib/Isothermal Liquid/Valves & Orifices/Orifices/Orifice (IL)  orifice_type=1  constant_orifice_spec=fluids.isothermal_liquid.valves_orifices.orifices.enum.constant_orifice_spec.area  variable_orifice_spec=fluids.isothermal_liquid.valves_orifices.orifices.enum.orifice_spec.linear  orifice_area_constant=2e-4 m^2  p_diff_TLU_constant=[-4, -3, -2, -1, -.5, 0, .5, 1, 2, 3, 4] MPa  vol_flow_TLU_constant=[-2.44, -2.12, -1.68, -1.22, -.84, 0, .85, 1.21, 1.7, 2.09, 2.41] .* 1e-3 m^3/s  S_min=0 m  del_S=5e-3 m  open_orientation=fluids.isothermal_liquid.valves_orifices.orifices.enum.orifice_orientation.positive  area_max=1e-4 m^2  area_leak=1e-10 m^2  S_TLU=[0, .002, .004, .007, .017] m  orifice_area_TLU=[1e-09, 2.0352e-07, 4.0736e-05, .00011438, .00034356] m^2  area=inf m^2  Cd=0.7  Re_c=150  smoothing_factor=0.01  pressure_recovery=false  S_vol_flow_TLU=[0, .002, .004, .007, .017] m  p_diff_TLU=[.3, .5, .7] MPa  vol_flow_TLU=1e-3 * [1.7e-05, 2e-05, 2.6e-05; .0035, .0045, .0053; .7, .9, 1.06; 1.96, 2.5, 3; 6, 7.7, 9.13] m^3/s
      settings: LibrarySourceBlock=sh_lib/Orifices/Fixed Orifice  InternalSimscapePortConfiguration="{\"Bottom\":[],\"Left\":[{\"id\":\"A\",\"label\":\"A\",\"type\":\"foundation.isothermal_liquid.isothermal_liquid\"}],\"Right\":[{\"id\":\"B\",\"label\":\"B\",\"type\":\"foundation.isothermal_liquid.isothermal_liquid\"}],\"Top\":[]}"
  Pressure Source : fl_lib/Isothermal Liquid/Sources/Pressure Source (IL)  source_type=1  pressure_differential=pOut_Init_WKSP bar
      settings: InternalSimscapePortConfiguration="{\"Bottom\":[],\"Left\":[{\"id\":\"A\",\"label\":\"A\",\"type\":\"foundation.isothermal_liquid.isothermal_liquid\"}],\"Right\":[{\"id\":\"B\",\"label\":\"B\",\"type\":\"foundation.isothermal_liquid.isothermal_liquid\"}],\"Top\":[]}"
      settings: LibrarySourceBlock=|
      | fl_lib/Hydraulic/Hydraulic Sources/Hydraulic Constant
      | Pressure Source
  A : PMIOPort  Side=Left
  B : PMIOPort  Port=2  Side=Right
  connections:
  Chamber/LConn1 -- Orifice/LConn1 -- A/RConn1
  Pressure Source/RConn1 -- Orifice/RConn1
  Pressure Source/LConn1 -- B/RConn1

== system sm_pump_triplex/Output Manifold ==
  Chamber : fl_lib/Isothermal Liquid/Elements/Constant Volume Chamber (IL)  volume=2e-4 m^3  p_I_specify=on  p_I_priority=High  p_I=pOut_Init_WKSP + 1.01325 bar  p_I_nominal_specify=off  p_I_nominal_value=1  p_I_nominal_unit=Pa
      settings: InternalSimscapePortConfiguration="{\"Bottom\":[],\"Left\":[{\"id\":\"A\",\"label\":\"A\",\"type\":\"foundation.isothermal_liquid.isothermal_liquid\"}],\"Right\":[],\"Top\":[]}"
      settings: LibrarySourceBlock=|
      | fl_lib/Hydraulic/Hydraulic Elements/Constant Volume
      | Hydraulic Chamber
  B : PMIOPort  Side=Right
  A1 : PMIOPort  Port=2  Side=Left
  A2 : PMIOPort  Port=3  Side=Left
  A3 : PMIOPort  Port=4  Side=Left
  connections:
  B/RConn1 -- Chamber/LConn1 -- A3/RConn1 -- A2/RConn1 -- A1/RConn1
